simulink model "hybrid_pv_wind_feeder"  (R2024b)
settings: Solver=FixedStepDiscrete  StartTime=0.0  StopTime=1.0  FixedStep=P.Ts  RelTol=1e-3
model workspace (MAT data in the model file):
  P : object (value not decoded)
symbols that are objects in the model workspace (value not decoded): P
undefined symbols (not defined in the file): DiscIntNeverNeededParam
libraries: spsThreePhaseSeriesRLCBranchLib x28, spsSeriesRLCBranchLib x14, spsThreePhaseParallelRLCLoadLib x12, spsIGBTDiodeLib x8, slpidlib x7, spsThreePhaseBreakerLib x6, simulink x4, spsGroundLib x4, spsThreePhaseVIMeasurementLib x4, spsControlledCurrentSourceLib x3, spsDiodeLib x2, spsAlphaBetaZerotodq0Lib x2
(part 1 of 2)
Description:
  | Hybrid PV-wind unit on the Pidari 400 V feeder (NEA, Janakpur DC).
  | Built by scripts/build_feeder_model.m from hybrid_pv_wind_islanding.slx and Real_model/nea_lv_feeder_data.m.
settings Model: LastModifiedBy=subas
settings SolverCC: AlgebraicLoopSolver=LineSearch
settings DataIOCC: ReturnWorkspaceOutputs=off
settings DebuggingCC: AlgebraicLoopMsg=none  ArithmeticOperatorsInVariantConditions=warning
settings ModelReferenceCC: EnableRefExpFcnMdlSchedulingChecks=on
settings SFSimCC: SimUseLocalCustomCode=off  CustomCodeUndefinedFunction=UseInterfaceOnly
settings RTWCC: RTWUseLocalCustomCode=off  GPUComputeCapability=3.5

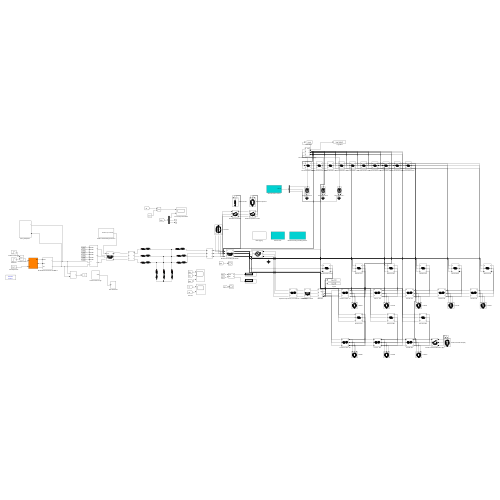
[thumbnail: Simulink's stored preview of the top-level diagram]
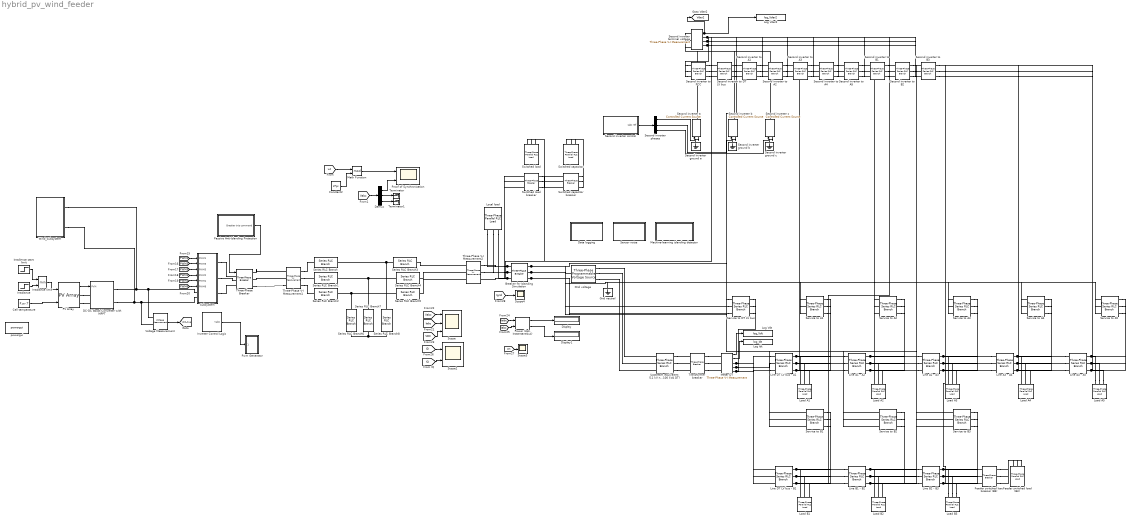
== system hybrid_pv_wind_feeder ==
  Breaker for Islanding Simulation : spsThreePhaseBreakerLib/Three-Phase Breaker  InitialState=closed  SwitchA=on  SwitchB=on  SwitchC=on  SwitchTimes=[P.tIsland]  External=off  BreakerResistance=0.01  SnubberResistance=1e6  SnubberCapacitance=inf  Measurements=None
  Cell temperature : Constant  Value=P.pv.T
  Constant2 : Constant  Value=2*pi
  DC-DC Boost Converter with MPPT : Subsystem
  Data logging : Subsystem
  Demux : Demux  Outputs=3
  Display : Display
  Display1 : Display
  Feeder switched load (B3) : spsThreePhaseParallelRLCLoadLib/Three-Phase Parallel RLC Load  LConnTagsString=A|B|C  Configuration=Y (grounded)  NominalVoltage=P.Vll  Vabc=[1e3 1e3 1e3]  Vabcp=[1e3 1e3 1e3]  NominalFrequency=P.fg  UnbalancedPower=off  ActivePower=P.feeder.swP  InductivePower=P.feeder.swQ  CapacitivePower=0  Pabc=[10e3 9e3 11e3]  QLabc=[100 90 110]  QCabc=[100 90 110]  Pabcp=[10e3 9e3 11e3]  QLabcp=[100 90 110]  QCabcp=[100 90 110]  Measurements=None  LoadType=constant Z
  Feeder switched load breaker (B3) : spsThreePhaseBreakerLib/Three-Phase Breaker  InitialState=open  SwitchA=on  SwitchB=on  SwitchC=on  SwitchTimes=[P.feeder.swT]  External=off  BreakerResistance=0.01  SnubberResistance=1e6  SnubberCapacitance=inf  Measurements=None
  Grid neutral : spsGroundLib/Ground  LConnTagsString=a
  Grid voltage : spsThreePhaseProgrammableVoltageSourceLib/Three-Phase Programmable Voltage Source  PositiveSequence=[P.feeder.Vsrc*P.Vll 0 P.fg]  VariationEntity=None  VariationType=Table of time-amplitude pairs  VariationTypeAlt=Step  VariationStep=P.event.step  VariationRate=P.event.rate  VariationMagnitude=0.3  VariationFrequency=2  VariationTiming=P.event.timing  VariationPhaseA=off  Amplitudes=P.event.amp  TimeValues=P.event.time  HarmonicGeneration=off  HarmonicA=P.grid.harmA  HarmonicB=P.grid.harmB  Timing=[0 1e6]  BusType=swing  Pref=0  Qref=0  Qmin=-inf  Qmax=inf
  Inverter Control Logic : Subsystem
  Irradiance : Step  Time=P.pv.tStep  Before=P.pv.G0  After=P.pv.G1  SampleTime=0
  Irradiance limit : MinMax  Inputs=2
  Irradiance start limit : Step  Time=P.pv.tStart  Before=P.pv.Gstart  After=1e4  SampleTime=0
  Line A1 - A2 : spsThreePhaseSeriesRLCBranchLib/Three-Phase Series RLC Branch  LConnTagsString=A|B|C  RConnTagsString=A|B|C  BranchType=RL  Resistance=P.feeder.lineR(2)  Inductance=P.feeder.lineL(2)  Capacitance=1e-6  Measurements=None
  Line A2 - A3 : spsThreePhaseSeriesRLCBranchLib/Three-Phase Series RLC Branch  LConnTagsString=A|B|C  RConnTagsString=A|B|C  BranchType=RL  Resistance=P.feeder.lineR(3)  Inductance=P.feeder.lineL(3)  Capacitance=1e-6  Measurements=None
  Line A3 - A4 : spsThreePhaseSeriesRLCBranchLib/Three-Phase Series RLC Branch  LConnTagsString=A|B|C  RConnTagsString=A|B|C  BranchType=RL  Resistance=P.feeder.lineR(4)  Inductance=P.feeder.lineL(4)  Capacitance=1e-6  Measurements=None
  Line A4 - A5 : spsThreePhaseSeriesRLCBranchLib/Three-Phase Series RLC Branch  LConnTagsString=A|B|C  RConnTagsString=A|B|C  BranchType=RL  Resistance=P.feeder.lineR(5)  Inductance=P.feeder.lineL(5)  Capacitance=1e-6  Measurements=None
  Line B1 - B2 : spsThreePhaseSeriesRLCBranchLib/Three-Phase Series RLC Branch  LConnTagsString=A|B|C  RConnTagsString=A|B|C  BranchType=RL  Resistance=P.feeder.lineR(7)  Inductance=P.feeder.lineL(7)  Capacitance=1e-6  Measurements=None
  Line B2 - B3 : spsThreePhaseSeriesRLCBranchLib/Three-Phase Series RLC Branch  LConnTagsString=A|B|C  RConnTagsString=A|B|C  BranchType=RL  Resistance=P.feeder.lineR(8)  Inductance=P.feeder.lineL(8)  Capacitance=1e-6  Measurements=None
  Line DT LV bus - A1 : spsThreePhaseSeriesRLCBranchLib/Three-Phase Series RLC Branch  LConnTagsString=A|B|C  RConnTagsString=A|B|C  BranchType=RL  Resistance=P.feeder.lineR(1)  Inductance=P.feeder.lineL(1)  Capacitance=1e-6  Measurements=None
  Line DT LV bus - B1 : spsThreePhaseSeriesRLCBranchLib/Three-Phase Series RLC Branch  LConnTagsString=A|B|C  RConnTagsString=A|B|C  BranchType=RL  Resistance=P.feeder.lineR(6)  Inductance=P.feeder.lineL(6)  Capacitance=1e-6  Measurements=None
  Load A1 : spsThreePhaseParallelRLCLoadLib/Three-Phase Parallel RLC Load  LConnTagsString=A|B|C  Configuration=Y (grounded)  NominalVoltage=P.Vll  Vabc=[1e3 1e3 1e3]  Vabcp=[1e3 1e3 1e3]  NominalFrequency=P.fg  UnbalancedPower=off  ActivePower=P.feeder.loadP(2)  InductivePower=P.feeder.loadQL(2)  CapacitivePower=0  Pabc=[10e3 9e3 11e3]  QLabc=[100 90 110]  QCabc=[100 90 110]  Pabcp=[10e3 9e3 11e3]  QLabcp=[100 90 110]  QCabcp=[100 90 110]  Measurements=None  LoadType=constant Z
  Load A2 : spsThreePhaseParallelRLCLoadLib/Three-Phase Parallel RLC Load  LConnTagsString=A|B|C  Configuration=Y (grounded)  NominalVoltage=P.Vll  Vabc=[1e3 1e3 1e3]  Vabcp=[1e3 1e3 1e3]  NominalFrequency=P.fg  UnbalancedPower=off  ActivePower=P.feeder.loadP(3)  InductivePower=P.feeder.loadQL(3)  CapacitivePower=0  Pabc=[10e3 9e3 11e3]  QLabc=[100 90 110]  QCabc=[100 90 110]  Pabcp=[10e3 9e3 11e3]  QLabcp=[100 90 110]  QCabcp=[100 90 110]  Measurements=None  LoadType=constant Z
  Load A3 : spsThreePhaseParallelRLCLoadLib/Three-Phase Parallel RLC Load  LConnTagsString=A|B|C  Configuration=Y (grounded)  NominalVoltage=P.Vll  Vabc=[1e3 1e3 1e3]  Vabcp=[1e3 1e3 1e3]  NominalFrequency=P.fg  UnbalancedPower=off  ActivePower=P.feeder.loadP(4)  InductivePower=P.feeder.loadQL(4)  CapacitivePower=0  Pabc=[10e3 9e3 11e3]  QLabc=[100 90 110]  QCabc=[100 90 110]  Pabcp=[10e3 9e3 11e3]  QLabcp=[100 90 110]  QCabcp=[100 90 110]  Measurements=None  LoadType=constant Z
  Load A4 : spsThreePhaseParallelRLCLoadLib/Three-Phase Parallel RLC Load  LConnTagsString=A|B|C  Configuration=Y (grounded)  NominalVoltage=P.Vll  Vabc=[1e3 1e3 1e3]  Vabcp=[1e3 1e3 1e3]  NominalFrequency=P.fg  UnbalancedPower=off  ActivePower=P.feeder.loadP(5)  InductivePower=P.feeder.loadQL(5)  CapacitivePower=0  Pabc=[10e3 9e3 11e3]  QLabc=[100 90 110]  QCabc=[100 90 110]  Pabcp=[10e3 9e3 11e3]  QLabcp=[100 90 110]  QCabcp=[100 90 110]  Measurements=None  LoadType=constant Z
  Load A5 : spsThreePhaseParallelRLCLoadLib/Three-Phase Parallel RLC Load  LConnTagsString=A|B|C  Configuration=Y (grounded)  NominalVoltage=P.Vll  Vabc=[1e3 1e3 1e3]  Vabcp=[1e3 1e3 1e3]  NominalFrequency=P.fg  UnbalancedPower=off  ActivePower=P.feeder.loadP(6)  InductivePower=P.feeder.loadQL(6)  CapacitivePower=0  Pabc=[10e3 9e3 11e3]  QLabc=[100 90 110]  QCabc=[100 90 110]  Pabcp=[10e3 9e3 11e3]  QLabcp=[100 90 110]  QCabcp=[100 90 110]  Measurements=None  LoadType=constant Z
  Load B1 : spsThreePhaseParallelRLCLoadLib/Three-Phase Parallel RLC Load  LConnTagsString=A|B|C  Configuration=Y (grounded)  NominalVoltage=P.Vll  Vabc=[1e3 1e3 1e3]  Vabcp=[1e3 1e3 1e3]  NominalFrequency=P.fg  UnbalancedPower=off  ActivePower=P.feeder.loadP(7)  InductivePower=P.feeder.loadQL(7)  CapacitivePower=0  Pabc=[10e3 9e3 11e3]  QLabc=[100 90 110]  QCabc=[100 90 110]  Pabcp=[10e3 9e3 11e3]  QLabcp=[100 90 110]  QCabcp=[100 90 110]  Measurements=None  LoadType=constant Z
  Load B2 : spsThreePhaseParallelRLCLoadLib/Three-Phase Parallel RLC Load  LConnTagsString=A|B|C  Configuration=Y (grounded)  NominalVoltage=P.Vll  Vabc=[1e3 1e3 1e3]  Vabcp=[1e3 1e3 1e3]  NominalFrequency=P.fg  UnbalancedPower=off  ActivePower=P.feeder.loadP(8)  InductivePower=P.feeder.loadQL(8)  CapacitivePower=0  Pabc=[10e3 9e3 11e3]  QLabc=[100 90 110]  QCabc=[100 90 110]  Pabcp=[10e3 9e3 11e3]  QLabcp=[100 90 110]  QCabcp=[100 90 110]  Measurements=None  LoadType=constant Z
  Load B3 : spsThreePhaseParallelRLCLoadLib/Three-Phase Parallel RLC Load  LConnTagsString=A|B|C  Configuration=Y (grounded)  NominalVoltage=P.Vll  Vabc=[1e3 1e3 1e3]  Vabcp=[1e3 1e3 1e3]  NominalFrequency=P.fg  UnbalancedPower=off  ActivePower=P.feeder.loadP(9)  InductivePower=P.feeder.loadQL(9)  CapacitivePower=0  Pabc=[10e3 9e3 11e3]  QLabc=[100 90 110]  QCabc=[100 90 110]  Pabcp=[10e3 9e3 11e3]  QLabcp=[100 90 110]  QCabcp=[100 90 110]  Measurements=None  LoadType=constant Z
  Local load : spsThreePhaseParallelRLCLoadLib/Three-Phase Parallel RLC Load  LConnTagsString=A|B|C  Configuration=Y (grounded)  NominalVoltage=P.Vll  Vabc=[1e3 1e3 1e3]  Vabcp=[1e3 1e3 1e3]  NominalFrequency=P.fg  UnbalancedPower=off  ActivePower=P.load.P  InductivePower=P.load.QL  CapacitivePower=P.load.QC  Pabc=[10e3 9e3 11e3]  QLabc=[100 90 110]  QCabc=[100 90 110]  Pabcp=[10e3 9e3 11e3]  QLabcp=[100 90 110]  QCabcp=[100 90 110]  Measurements=None  LoadType=constant Z
  Log Idt : ToWorkspace  VariableName=log_Idt  SaveFormat=Timeseries  SampleTime=-1
      settings: Decimation=P.logDecim
  Log Vder2 : ToWorkspace  VariableName=log_Vder2  SaveFormat=Timeseries  SampleTime=-1
      settings: Decimation=P.logDecim
  Log Vdt : ToWorkspace  VariableName=log_Vdt  SaveFormat=Timeseries  SampleTime=-1
      settings: Decimation=P.logDecim
  Machine-learning islanding detector : Subsystem
  Math Function : Math  Operator=mod  SignedPower=on
  Meter DT : spsThreePhaseVIMeasurementLib/Three-Phase V-I Measurement  VoltageMeasurement=phase-to-ground  SetLabelV=off  LabelV=Vabc  Vpu=off  VpuLL=off  CurrentMeasurement=yes  SetLabelI=off  LabelI=Iabc  Ipu=off  Pbase=100e6  Vbase=500e3  OutputType=Complex  PhasorSimulation=off  PSBequivalent=0
  PV Array : spsPVArrayLib/PV Array  Npar=P.pv.Npar  Nser=P.pv.Nser  PlotType=array @ 1000 W/m2 & specified temperatures  S_vec="[ 1000  500  100 ]"  Temp_C_vec="[ 45 25  ]"  ModuleName=User-defined  PlotWhenSelected=off  Pm=213.15  Ncell=60  Voc=36.3  Isc=7.84  Vm=29  Im=7.35  beta_Voc_pc=-0.36099  alpha_Isc_pc=0.102  beta_Voc=-0.13104  alpha_Isc=0.0079968  IL=7.8654  I0=2.9273e-10  nI=0.98119  Rsh=313.0553  Rs=0.39381  RobustModel=off  RobustCellTemperature=313.3991  BAL=on  Tc=1e-6  Tfilter=5e-5
  Passive Anti-Islanding Protection : Subsystem
  "Power (3ph, Instantaneous)" : spsPower3phInstantaneousLib/Power (3ph, Instantaneous)
  Proof of Synchronization : Scope  NumInputPorts=2
  "Pwm Generator " : Subsystem
  Scope : Scope  NumInputPorts=3
  Scope2 : Scope  NumInputPorts=2
  Scope3 : Scope
  Scope4 : Scope
  Second inverter a : spsControlledCurrentSourceLib/Controlled Current Source  Initialize=off  Source_Type=AC  Amplitude=0  Phase=0  Frequency=0  Measurements=None
  Second inverter b : spsControlledCurrentSourceLib/Controlled Current Source  Initialize=off  Source_Type=AC  Amplitude=0  Phase=0  Frequency=0  Measurements=None
  Second inverter c : spsControlledCurrentSourceLib/Controlled Current Source  Initialize=off  Source_Type=AC  Amplitude=0  Phase=0  Frequency=0  Measurements=None
  Second inverter control : Subsystem
  Second inverter ground a : spsGroundLib/Ground  LConnTagsString=a
  Second inverter ground b : spsGroundLib/Ground  LConnTagsString=a
  Second inverter ground c : spsGroundLib/Ground  LConnTagsString=a
  Second inverter phases : Demux  Outputs=3
  Second inverter terminal voltage : spsThreePhaseVIMeasurementLib/Three-Phase V-I Measurement  VoltageMeasurement=phase-to-ground  SetLabelV=off  LabelV=Vabc  Vpu=off  VpuLL=off  CurrentMeasurement=no  SetLabelI=off  LabelI=Iabc  Ipu=off  Pbase=100e6  Vbase=500e3  OutputType=Complex  PhasorSimulation=off  PSBequivalent=0
  Second inverter to A1 : spsThreePhaseSeriesRLCBranchLib/Three-Phase Series RLC Branch  LConnTagsString=A|B|C  RConnTagsString=A|B|C  BranchType=R  Resistance=P.feeder.rDer2(3)  Inductance=1e-3  Capacitance=1e-6  Measurements=None
  Second inverter to A2 : spsThreePhaseSeriesRLCBranchLib/Three-Phase Series RLC Branch  LConnTagsString=A|B|C  RConnTagsString=A|B|C  BranchType=R  Resistance=P.feeder.rDer2(4)  Inductance=1e-3  Capacitance=1e-6  Measurements=None
  Second inverter to A3 : spsThreePhaseSeriesRLCBranchLib/Three-Phase Series RLC Branch  LConnTagsString=A|B|C  RConnTagsString=A|B|C  BranchType=R  Resistance=P.feeder.rDer2(5)  Inductance=1e-3  Capacitance=1e-6  Measurements=None
  Second inverter to A4 : spsThreePhaseSeriesRLCBranchLib/Three-Phase Series RLC Branch  LConnTagsString=A|B|C  RConnTagsString=A|B|C  BranchType=R  Resistance=P.feeder.rDer2(6)  Inductance=1e-3  Capacitance=1e-6  Measurements=None
  Second inverter to A5 : spsThreePhaseSeriesRLCBranchLib/Three-Phase Series RLC Branch  LConnTagsString=A|B|C  RConnTagsString=A|B|C  BranchType=R  Resistance=P.feeder.rDer2(7)  Inductance=1e-3  Capacitance=1e-6  Measurements=None
  Second inverter to B1 : spsThreePhaseSeriesRLCBranchLib/Three-Phase Series RLC Branch  LConnTagsString=A|B|C  RConnTagsString=A|B|C  BranchType=R  Resistance=P.feeder.rDer2(8)  Inductance=1e-3  Capacitance=1e-6  Measurements=None
  Second inverter to B2 : spsThreePhaseSeriesRLCBranchLib/Three-Phase Series RLC Branch  LConnTagsString=A|B|C  RConnTagsString=A|B|C  BranchType=R  Resistance=P.feeder.rDer2(9)  Inductance=1e-3  Capacitance=1e-6  Measurements=None
  Second inverter to B3 : spsThreePhaseSeriesRLCBranchLib/Three-Phase Series RLC Branch  LConnTagsString=A|B|C  RConnTagsString=A|B|C  BranchType=R  Resistance=P.feeder.rDer2(10)  Inductance=1e-3  Capacitance=1e-6  Measurements=None
  Second inverter to DT LV bus : spsThreePhaseSeriesRLCBranchLib/Three-Phase Series RLC Branch  LConnTagsString=A|B|C  RConnTagsString=A|B|C  BranchType=R  Resistance=P.feeder.rDer2(2)  Inductance=1e-3  Capacitance=1e-6  Measurements=None
  Second inverter to PCC : spsThreePhaseSeriesRLCBranchLib/Three-Phase Series RLC Branch  LConnTagsString=A|B|C  RConnTagsString=A|B|C  BranchType=R  Resistance=P.feeder.rDer2(1)  Inductance=1e-3  Capacitance=1e-6  Measurements=None
  Sensor noise : Subsystem
  Series RLC Branch : spsSeriesRLCBranchLib/Series RLC Branch  LConnTagsString=__new0  RConnTagsString=__new0  BranchType=RL  Resistance=P.lcl.R1  Inductance=P.lcl.L1  SetiL0=off  InitialCurrent=0  Capacitance=1e-6  Setx0=off  InitialVoltage=0  Measurements=None
  Series RLC Branch1 : spsSeriesRLCBranchLib/Series RLC Branch  LConnTagsString=__new0  RConnTagsString=__new0  BranchType=RL  Resistance=P.lcl.R1  Inductance=P.lcl.L1  SetiL0=off  InitialCurrent=0  Capacitance=1e-6  Setx0=off  InitialVoltage=0  Measurements=None
  Series RLC Branch2 : spsSeriesRLCBranchLib/Series RLC Branch  LConnTagsString=__new0  RConnTagsString=__new0  BranchType=RL  Resistance=P.lcl.R1  Inductance=P.lcl.L1  SetiL0=off  InitialCurrent=0  Capacitance=1e-6  Setx0=off  InitialVoltage=0  Measurements=None
  Series RLC Branch3 : spsSeriesRLCBranchLib/Series RLC Branch  LConnTagsString=__new0  RConnTagsString=__new0  BranchType=RL  Resistance=P.lcl.R2  Inductance=P.lcl.L2  SetiL0=off  InitialCurrent=10  Capacitance=1e-6  Setx0=off  InitialVoltage=0  Measurements=None
  Series RLC Branch4 : spsSeriesRLCBranchLib/Series RLC Branch  LConnTagsString=__new0  RConnTagsString=__new0  BranchType=RL  Resistance=P.lcl.R2  Inductance=P.lcl.L2  SetiL0=off  InitialCurrent=10  Capacitance=1e-6  Setx0=off  InitialVoltage=0  Measurements=None
  Series RLC Branch5 : spsSeriesRLCBranchLib/Series RLC Branch  LConnTagsString=__new0  RConnTagsString=__new0  BranchType=RL  Resistance=P.lcl.R2  Inductance=P.lcl.L2  SetiL0=off  InitialCurrent=10  Capacitance=1e-6  Setx0=off  InitialVoltage=0  Measurements=None
  Series RLC Branch6 : spsSeriesRLCBranchLib/Series RLC Branch  LConnTagsString=__new0  RConnTagsString=__new0  BranchType=RC  Resistance=P.lcl.Rd  Inductance=1000e-3  SetiL0=off  InitialCurrent=0  Capacitance=P.lcl.Cf  Setx0=off  InitialVoltage=0  Measurements=None
  Series RLC Branch7 : spsSeriesRLCBranchLib/Series RLC Branch  LConnTagsString=__new0  RConnTagsString=__new0  BranchType=RC  Resistance=P.lcl.Rd  Inductance=1000e-3  SetiL0=off  InitialCurrent=0  Capacitance=P.lcl.Cf  Setx0=off  InitialVoltage=0  Measurements=None
  Series RLC Branch8 : spsSeriesRLCBranchLib/Series RLC Branch  LConnTagsString=__new0  RConnTagsString=__new0  BranchType=RC  Resistance=P.lcl.Rd  Inductance=1000e-3  SetiL0=off  InitialCurrent=0  Capacitance=P.lcl.Cf  Setx0=off  InitialVoltage=0  Measurements=None
  Service to A1 : spsThreePhaseSeriesRLCBranchLib/Three-Phase Series RLC Branch  LConnTagsString=A|B|C  RConnTagsString=A|B|C  BranchType=R  Resistance=P.feeder.rConn(2)  Inductance=1e-3  Capacitance=1e-6  Measurements=None
  Service to A2 : spsThreePhaseSeriesRLCBranchLib/Three-Phase Series RLC Branch  LConnTagsString=A|B|C  RConnTagsString=A|B|C  BranchType=R  Resistance=P.feeder.rConn(3)  Inductance=1e-3  Capacitance=1e-6  Measurements=None
  Service to A3 : spsThreePhaseSeriesRLCBranchLib/Three-Phase Series RLC Branch  LConnTagsString=A|B|C  RConnTagsString=A|B|C  BranchType=R  Resistance=P.feeder.rConn(4)  Inductance=1e-3  Capacitance=1e-6  Measurements=None
  Service to A4 : spsThreePhaseSeriesRLCBranchLib/Three-Phase Series RLC Branch  LConnTagsString=A|B|C  RConnTagsString=A|B|C  BranchType=R  Resistance=P.feeder.rConn(5)  Inductance=1e-3  Capacitance=1e-6  Measurements=None
  Service to A5 : spsThreePhaseSeriesRLCBranchLib/Three-Phase Series RLC Branch  LConnTagsString=A|B|C  RConnTagsString=A|B|C  BranchType=R  Resistance=P.feeder.rConn(6)  Inductance=1e-3  Capacitance=1e-6  Measurements=None
  Service to B1 : spsThreePhaseSeriesRLCBranchLib/Three-Phase Series RLC Branch  LConnTagsString=A|B|C  RConnTagsString=A|B|C  BranchType=R  Resistance=P.feeder.rConn(7)  Inductance=1e-3  Capacitance=1e-6  Measurements=None
  Service to B2 : spsThreePhaseSeriesRLCBranchLib/Three-Phase Series RLC Branch  LConnTagsString=A|B|C  RConnTagsString=A|B|C  BranchType=R  Resistance=P.feeder.rConn(8)  Inductance=1e-3  Capacitance=1e-6  Measurements=None
  Service to B3 : spsThreePhaseSeriesRLCBranchLib/Three-Phase Series RLC Branch  LConnTagsString=A|B|C  RConnTagsString=A|B|C  BranchType=R  Resistance=P.feeder.rConn(9)  Inductance=1e-3  Capacitance=1e-6  Measurements=None
  Service to DT LV bus : spsThreePhaseSeriesRLCBranchLib/Three-Phase Series RLC Branch  LConnTagsString=A|B|C  RConnTagsString=A|B|C  BranchType=R  Resistance=P.feeder.rConn(1)  Inductance=1e-3  Capacitance=1e-6  Measurements=None
  Subsystem : Subsystem
  Switched capacitor : spsThreePhaseParallelRLCLoadLib/Three-Phase Parallel RLC Load  LConnTagsString=A|B|C  Configuration=Y (grounded)  NominalVoltage=P.Vll  Vabc=[1e3 1e3 1e3]  Vabcp=[1e3 1e3 1e3]  NominalFrequency=P.fg  UnbalancedPower=off  ActivePower=1  InductivePower=0  CapacitivePower=P.event.capQ  Pabc=[10e3 9e3 11e3]  QLabc=[100 90 110]  QCabc=[100 90 110]  Pabcp=[10e3 9e3 11e3]  QLabcp=[100 90 110]  QCabcp=[100 90 110]  Measurements=None  LoadType=constant Z
  Switched capacitor breaker : spsThreePhaseBreakerLib/Three-Phase Breaker  InitialState=open  SwitchA=on  SwitchB=on  SwitchC=on  SwitchTimes=[P.event.capT]  External=off  BreakerResistance=0.01  SnubberResistance=1e6  SnubberCapacitance=inf  Measurements=None
  Switched load : spsThreePhaseParallelRLCLoadLib/Three-Phase Parallel RLC Load  LConnTagsString=A|B|C  Configuration=Y (grounded)  NominalVoltage=P.Vll  Vabc=[1e3 1e3 1e3]  Vabcp=[1e3 1e3 1e3]  NominalFrequency=P.fg  UnbalancedPower=off  ActivePower=P.event.loadP  InductivePower=0  CapacitivePower=0  Pabc=[10e3 9e3 11e3]  QLabc=[100 90 110]  QCabc=[100 90 110]  Pabcp=[10e3 9e3 11e3]  QLabcp=[100 90 110]  QCabcp=[100 90 110]  Measurements=None  LoadType=constant Z
  Switched load breaker : spsThreePhaseBreakerLib/Three-Phase Breaker  InitialState=open  SwitchA=on  SwitchB=on  SwitchC=on  SwitchTimes=[P.event.loadT]  External=off  BreakerResistance=0.01  SnubberResistance=1e6  SnubberCapacitance=inf  Measurements=None
  Terminator : Terminator
  Terminator1 : Terminator
  Three-Phase V-I Measurement1 : spsThreePhaseVIMeasurementLib/Three-Phase V-I Measurement  VoltageMeasurement=no  SetLabelV=off  LabelV=Vabc  Vpu=off  VpuLL=off  CurrentMeasurement=yes  SetLabelI=on  LabelI=Iabc_true  Ipu=off  Pbase=100e6  Vbase=500e3  OutputType=Complex  PhasorSimulation=off  PSBequivalent=0
  Three-Phase V-I Measurement2 : spsThreePhaseVIMeasurementLib/Three-Phase V-I Measurement  VoltageMeasurement=phase-to-ground  SetLabelV=on  LabelV=Vabc_true  Vpu=off  VpuLL=off  CurrentMeasurement=yes  SetLabelI=on  LabelI=Igrid_true  Ipu=off  Pbase=100e6  Vbase=500e3  OutputType=Complex  PhasorSimulation=off  PSBequivalent=0
  Three-Phase Breaker : spsThreePhaseBreakerLib/Three-Phase Breaker  InitialState=closed  SwitchA=on  SwitchB=on  SwitchC=on  SwitchTimes=[9999]  External=on  BreakerResistance=0.01  SnubberResistance=1e6  SnubberCapacitance=inf  Measurements=None
  Transformer breaker : spsThreePhaseBreakerLib/Three-Phase Breaker  InitialState=closed  SwitchA=on  SwitchB=on  SwitchC=on  SwitchTimes=[P.feeder.tIsland]  External=off  BreakerResistance=0.01  SnubberResistance=1e6  SnubberCapacitance=inf  Measurements=None
  Upstream equivalent (11 kV network + 100 kVA DT) : spsThreePhaseSeriesRLCBranchLib/Three-Phase Series RLC Branch  LConnTagsString=A|B|C  RConnTagsString=A|B|C  BranchType=RL  Resistance=P.feeder.Rsrc  Inductance=P.feeder.Lsrc  Capacitance=1e-6  Measurements=None
  Voltage Measurement : spsVoltageMeasurementLib/Voltage Measurement  PhasorSimulation=off  OutputType=Complex  PSBequivalent=0
  Wind_Subsystem : Subsystem
  powergui : spspowerguiLib/powergui  Priority=1  SimulationMode=Discrete  SampleTime=P.Ts  frequency=60  Iterations=50  frequencyindice=0  Pbase=100e6  ErrMax=1e-4  UnitsV=kV  UnitsW=MW  buscounter=0  FunctionMessages=off  echomessages=off  EnableUseOfTLC=off  CurrentSourceSwitches=off  DisableSnubberDevices=off  DisableRonSwitches=off  DisableVfSwitches=off  DisplayEquations=off  AutomaticDiscreteSolvers=off  SolverType=Tustin/Backward Euler (TBE)  Interpol=off  ExternalGateDelay=off  methode=off  Ts=100  x0status=blocks  SPID=off  SwTol=0  HookPort=off  NonlinearTolerance=1e-4  nMaxIteration=100  ContinueOnMaxIteration=off  RestoreLinks=warning  ResistiveCurrentMeasurement=off  Frange=[0:2:500]  Ylog=off  Xlog=on  ShowGrid=off  save=off  variable=ZData  structure=Grid_current  ZoomFFT=off  StartTime=0.4  cycles=5  DisplayStyle=1  fundamental=50  FreqAxis=off  MaxFrequency=1000  frequencyindicesteady=1  RmsSteady=1  display=off
  tag scope: VDC_true=global, Vder2=global
  wires:
  Voltage Measurement/1 -> [VDC_true]
  [PWM6] -> Subsystem/6(PWM6)
  [PWM1] -> Subsystem/1(PWM1)
  "Power (3ph, Instantaneous)"/1 -> Display/1
  PV Array/1 -> DC-DC Boost Converter with MPPT/1("PVM ")
  [Iabc] -> "Power (3ph, Instantaneous)"/2
  [PWM3] -> Subsystem/2(PWM3)
  [Igrid] -> Scope4/1
  Inverter Control Logic/1(Vabc) -> "Pwm Generator "/1(1)
  [PWM4] -> Subsystem/5(PWM4)
  [Vabc] -> Scope/1
  [Vabc] -> "Power (3ph, Instantaneous)"/1
  [ID] -> Scope2/1
  "Power (3ph, Instantaneous)"/2 -> Display1/1
  [wt] -> Scope3/1
  [PWM2] -> Subsystem/4(PWM2)
  [VDC] -> Scope/3
  [PWM5] -> Subsystem/3(PWM5)
  [Iabc] -> Scope/2
  Passive Anti-Islanding Protection/1("Breaker trip command ") -> Three-Phase Breaker/1
  Demux/1 -> Proof of Synchronization/2
  Demux/2 -> Terminator/1
  Constant2/1 -> Math Function/2
  [wt] -> Math Function/1
  Math Function/1 -> Proof of Synchronization/1
  [Vabc] -> Demux/1
  Demux/3 -> Terminator1/1
  Irradiance/1 -> Irradiance limit/2
  Irradiance start limit/1 -> Irradiance limit/1
  Irradiance limit/1 -> PV Array/1
  Cell temperature/1 -> PV Array/2
  Second inverter control/1(Iabc ref) -> Second inverter phases/1
  Second inverter phases/1 -> Second inverter a/1
  Second inverter phases/2 -> Second inverter b/1
  Second inverter phases/3 -> Second inverter c/1
  [IQ] -> Scope2/2
  Meter DT/1 -> Log Vdt/1
  Meter DT/2 -> Log Idt/1
  Second inverter terminal voltage/1 -> [Vder2], Log Vder2/1
  connections:
  Series RLC Branch7/RConn1 -- Series RLC Branch8/RConn1 -- Series RLC Branch6/RConn1
  Series RLC Branch8/LConn1 -- Series RLC Branch/RConn1 -- Series RLC Branch3/LConn1
  Series RLC Branch7/LConn1 -- Series RLC Branch1/RConn1 -- Series RLC Branch4/LConn1
  Series RLC Branch6/LConn1 -- Series RLC Branch2/RConn1 -- Series RLC Branch5/LConn1
  PV Array/RConn1 -- DC-DC Boost Converter with MPPT/LConn1
  Three-Phase V-I Measurement1/RConn3 -- Series RLC Branch2/LConn1
  Three-Phase V-I Measurement1/RConn1 -- Series RLC Branch/LConn1
  PV Array/RConn2 -- DC-DC Boost Converter with MPPT/LConn2
  Three-Phase V-I Measurement1/RConn2 -- Series RLC Branch1/LConn1
  DC-DC Boost Converter with MPPT/RConn1 -- Wind_Subsystem/RConn1 -- Subsystem/LConn1 -- Voltage Measurement/LConn1
  DC-DC Boost Converter with MPPT/RConn2 -- Wind_Subsystem/RConn2 -- Subsystem/LConn2 -- Voltage Measurement/LConn2
  Subsystem/RConn1 -- Three-Phase Breaker/LConn1
  Subsystem/RConn2 -- Three-Phase Breaker/LConn2
  Subsystem/RConn3 -- Three-Phase Breaker/LConn3
  Three-Phase Breaker/RConn1 -- Three-Phase V-I Measurement1/LConn1
  Three-Phase V-I Measurement1/LConn2 -- Three-Phase Breaker/RConn2
  Three-Phase Breaker/RConn3 -- Three-Phase V-I Measurement1/LConn3
  Three-Phase V-I Measurement2/LConn1 -- Local load/LConn1 -- Switched load breaker/LConn1 -- Switched capacitor breaker/LConn1 -- Breaker for Islanding Simulation/LConn1 -- Second inverter to PCC/RConn1
  Three-Phase V-I Measurement2/LConn2 -- Local load/LConn2 -- Switched load breaker/LConn2 -- Switched capacitor breaker/LConn2 -- Breaker for Islanding Simulation/LConn2 -- Second inverter to PCC/RConn2
  Three-Phase V-I Measurement2/LConn3 -- Breaker for Islanding Simulation/LConn3 -- Local load/LConn3 -- Switched load breaker/LConn3 -- Switched capacitor breaker/LConn3 -- Second inverter to PCC/RConn3
  Series RLC Branch3/RConn1 -- Three-Phase V-I Measurement2/RConn1
  Series RLC Branch4/RConn1 -- Three-Phase V-I Measurement2/RConn2
  Series RLC Branch5/RConn1 -- Three-Phase V-I Measurement2/RConn3
  Grid voltage/LConn1 -- Grid neutral/LConn1
  Switched load breaker/RConn1 -- Switched load/LConn1
  Switched load breaker/RConn2 -- Switched load/LConn2
  Switched load breaker/RConn3 -- Switched load/LConn3
  Switched capacitor breaker/RConn1 -- Switched capacitor/LConn1
  Switched capacitor breaker/RConn2 -- Switched capacitor/LConn2
  Switched capacitor breaker/RConn3 -- Switched capacitor/LConn3
  Second inverter a/LConn1 -- Second inverter ground a/LConn1
  Second inverter b/LConn1 -- Second inverter ground b/LConn1
  Second inverter c/LConn1 -- Second inverter ground c/LConn1
  Grid voltage/RConn1 -- Upstream equivalent (11 kV network + 100 kVA DT)/LConn1
  Grid voltage/RConn2 -- Upstream equivalent (11 kV network + 100 kVA DT)/LConn2
  Grid voltage/RConn3 -- Upstream equivalent (11 kV network + 100 kVA DT)/LConn3
  Upstream equivalent (11 kV network + 100 kVA DT)/RConn1 -- Transformer breaker/LConn1
  Upstream equivalent (11 kV network + 100 kVA DT)/RConn2 -- Transformer breaker/LConn2
  Upstream equivalent (11 kV network + 100 kVA DT)/RConn3 -- Transformer breaker/LConn3
  Transformer breaker/RConn1 -- Meter DT/LConn1
  Transformer breaker/RConn2 -- Meter DT/LConn2
  Transformer breaker/RConn3 -- Meter DT/LConn3
  Line DT LV bus - A1/LConn1 -- Meter DT/RConn1 -- Line DT LV bus - B1/LConn1 -- Service to DT LV bus/RConn1 -- Second inverter to DT LV bus/RConn1
  Line DT LV bus - A1/LConn2 -- Meter DT/RConn2 -- Line DT LV bus - B1/LConn2 -- Service to DT LV bus/RConn2 -- Second inverter to DT LV bus/RConn2
  Line DT LV bus - A1/LConn3 -- Meter DT/RConn3 -- Line DT LV bus - B1/LConn3 -- Service to DT LV bus/RConn3 -- Second inverter to DT LV bus/RConn3
  Line A1 - A2/LConn1 -- Line DT LV bus - A1/RConn1 -- Load A1/LConn1 -- Service to A1/RConn1 -- Second inverter to A1/RConn1
  Line A1 - A2/LConn2 -- Line DT LV bus - A1/RConn2 -- Load A1/LConn2 -- Service to A1/RConn2 -- Second inverter to A1/RConn2
  Line A1 - A2/LConn3 -- Line DT LV bus - A1/RConn3 -- Load A1/LConn3 -- Service to A1/RConn3 -- Second inverter to A1/RConn3
  Line A2 - A3/LConn1 -- Line A1 - A2/RConn1 -- Load A2/LConn1 -- Service to A2/RConn1 -- Second inverter to A2/RConn1
  Line A2 - A3/LConn2 -- Line A1 - A2/RConn2 -- Load A2/LConn2 -- Service to A2/RConn2 -- Second inverter to A2/RConn2
  Line A2 - A3/LConn3 -- Line A1 - A2/RConn3 -- Load A2/LConn3 -- Service to A2/RConn3 -- Second inverter to A2/RConn3
  Line A3 - A4/LConn1 -- Line A2 - A3/RConn1 -- Load A3/LConn1 -- Service to A3/RConn1 -- Second inverter to A3/RConn1
  Line A3 - A4/LConn2 -- Line A2 - A3/RConn2 -- Load A3/LConn2 -- Service to A3/RConn2 -- Second inverter to A3/RConn2
  Line A3 - A4/LConn3 -- Line A2 - A3/RConn3 -- Load A3/LConn3 -- Service to A3/RConn3 -- Second inverter to A3/RConn3
  Line A4 - A5/LConn1 -- Line A3 - A4/RConn1 -- Load A4/LConn1 -- Service to A4/RConn1 -- Second inverter to A4/RConn1
  Line A4 - A5/LConn2 -- Line A3 - A4/RConn2 -- Load A4/LConn2 -- Service to A4/RConn2 -- Second inverter to A4/RConn2
  Line A4 - A5/LConn3 -- Line A3 - A4/RConn3 -- Load A4/LConn3 -- Service to A4/RConn3 -- Second inverter to A4/RConn3
  Line B1 - B2/LConn1 -- Line DT LV bus - B1/RConn1 -- Load B1/LConn1 -- Service to B1/RConn1 -- Second inverter to B1/RConn1
  Line B1 - B2/LConn2 -- Line DT LV bus - B1/RConn2 -- Load B1/LConn2 -- Service to B1/RConn2 -- Second inverter to B1/RConn2
  Line B1 - B2/LConn3 -- Line DT LV bus - B1/RConn3 -- Load B1/LConn3 -- Service to B1/RConn3 -- Second inverter to B1/RConn3
  Line B2 - B3/LConn1 -- Line B1 - B2/RConn1 -- Load B2/LConn1 -- Service to B2/RConn1 -- Second inverter to B2/RConn1
  Line B2 - B3/LConn2 -- Line B1 - B2/RConn2 -- Load B2/LConn2 -- Service to B2/RConn2 -- Second inverter to B2/RConn2
  Line B2 - B3/LConn3 -- Line B1 - B2/RConn3 -- Load B2/LConn3 -- Service to B2/RConn3 -- Second inverter to B2/RConn3
  Load A5/LConn1 -- Line A4 - A5/RConn1 -- Service to A5/RConn1 -- Second inverter to A5/RConn1
  Load A5/LConn2 -- Line A4 - A5/RConn2 -- Service to A5/RConn2 -- Second inverter to A5/RConn2
  Load A5/LConn3 -- Line A4 - A5/RConn3 -- Service to A5/RConn3 -- Second inverter to A5/RConn3
  Load B3/LConn1 -- Line B2 - B3/RConn1 -- Feeder switched load breaker (B3)/LConn1 -- Service to B3/RConn1 -- Second inverter to B3/RConn1
  Load B3/LConn2 -- Line B2 - B3/RConn2 -- Feeder switched load breaker (B3)/LConn2 -- Service to B3/RConn2 -- Second inverter to B3/RConn2
  Load B3/LConn3 -- Line B2 - B3/RConn3 -- Feeder switched load breaker (B3)/LConn3 -- Service to B3/RConn3 -- Second inverter to B3/RConn3
  Feeder switched load breaker (B3)/RConn1 -- Feeder switched load (B3)/LConn1
  Feeder switched load breaker (B3)/RConn2 -- Feeder switched load (B3)/LConn2
  Feeder switched load breaker (B3)/RConn3 -- Feeder switched load (B3)/LConn3
  Service to DT LV bus/LConn1 -- Breaker for Islanding Simulation/RConn1 -- Service to A1/LConn1 -- Service to A2/LConn1 -- Service to A3/LConn1 -- Service to A4/LConn1 -- Service to A5/LConn1 -- Service to B1/LConn1 -- Service to B2/LConn1 -- Service to B3/LConn1
  Service to DT LV bus/LConn2 -- Breaker for Islanding Simulation/RConn2 -- Service to A1/LConn2 -- Service to A2/LConn2 -- Service to A3/LConn2 -- Service to A4/LConn2 -- Service to A5/LConn2 -- Service to B1/LConn2 -- Service to B2/LConn2 -- Service to B3/LConn2
  Service to DT LV bus/LConn3 -- Breaker for Islanding Simulation/RConn3 -- Service to A1/LConn3 -- Service to A2/LConn3 -- Service to A3/LConn3 -- Service to A4/LConn3 -- Service to A5/LConn3 -- Service to B1/LConn3 -- Service to B2/LConn3 -- Service to B3/LConn3
  Second inverter a/RConn1 -- Second inverter terminal voltage/LConn1
  Second inverter b/RConn1 -- Second inverter terminal voltage/LConn2
  Second inverter c/RConn1 -- Second inverter terminal voltage/LConn3
  Second inverter to PCC/LConn1 -- Second inverter terminal voltage/RConn1 -- Second inverter to DT LV bus/LConn1 -- Second inverter to A1/LConn1 -- Second inverter to A2/LConn1 -- Second inverter to A3/LConn1 -- Second inverter to A4/LConn1 -- Second inverter to A5/LConn1 -- Second inverter to B1/LConn1 -- Second inverter to B2/LConn1 -- Second inverter to B3/LConn1
  Second inverter to PCC/LConn2 -- Second inverter terminal voltage/RConn2 -- Second inverter to DT LV bus/LConn2 -- Second inverter to A1/LConn2 -- Second inverter to A2/LConn2 -- Second inverter to A3/LConn2 -- Second inverter to A4/LConn2 -- Second inverter to A5/LConn2 -- Second inverter to B1/LConn2 -- Second inverter to B2/LConn2 -- Second inverter to B3/LConn2
  Second inverter to PCC/LConn3 -- Second inverter terminal voltage/RConn3 -- Second inverter to DT LV bus/LConn3 -- Second inverter to A1/LConn3 -- Second inverter to A2/LConn3 -- Second inverter to A3/LConn3 -- Second inverter to A4/LConn3 -- Second inverter to A5/LConn3 -- Second inverter to B1/LConn3 -- Second inverter to B2/LConn3 -- Second inverter to B3/LConn3

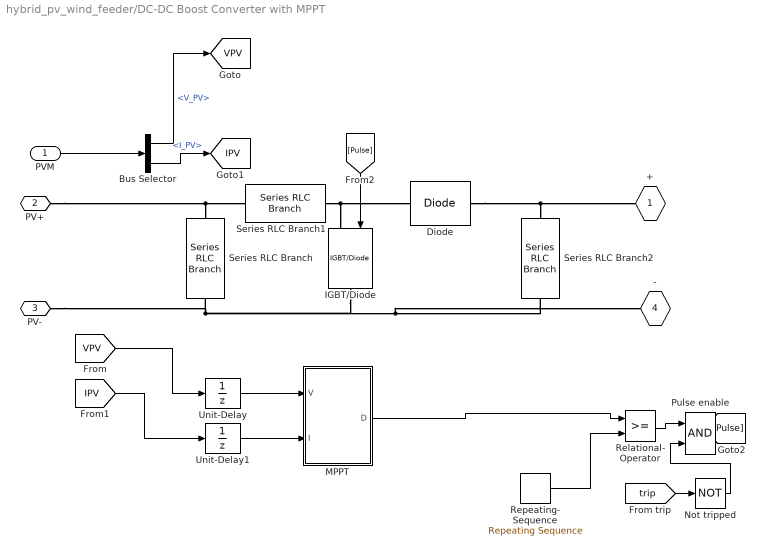
== system hybrid_pv_wind_feeder/DC-DC Boost Converter with MPPT ==
  "PVM " : Inport
  Bus Selector : BusSelector  OutputSignals=V_PV,I_PV
  Diode : spsDiodeLib/Diode  Ron=0.001  Lon=0  Vf=0.8  IC=0  UseSnubber=0  Rs=500  Cs=250e-9  Measurements=off
  IGBT/Diode : spsIGBTDiodeLib/IGBT//Diode  Ron=1e-3  Rs=1e5  Cs=inf  Measurements=off
  MPPT : MATLAB Function  TreatAsAtomicUnit=on
  Not tripped : Logic  Operator=NOT  AllPortsSameDT=off  OutDataTypeStr=boolean
  Pulse enable : Logic  AllPortsSameDT=off  OutDataTypeStr=boolean
  Relational- Operator : RelationalOperator  OutDataTypeStr=boolean  RndMeth=Simplest  InputSameDT=off
  Repeating- Sequence : simulink/Sources/Repeating Sequence  rep_seq_t=[0 0.0002]  rep_seq_y=[0 1]
  Series RLC Branch : spsSeriesRLCBranchLib/Series RLC Branch  LConnTagsString=__new0  RConnTagsString=__new0  BranchType=RC  Resistance=1e-3  Inductance=1e-3  SetiL0=off  InitialCurrent=0  Capacitance=1000e-6  Setx0=off  InitialVoltage=0  Measurements=None
  Series RLC Branch1 : spsSeriesRLCBranchLib/Series RLC Branch  LConnTagsString=__new0  RConnTagsString=__new0  BranchType=L  Resistance=1e-3  Inductance=1.5e-3  SetiL0=off  InitialCurrent=0  Capacitance=1000e-6  Setx0=off  InitialVoltage=0  Measurements=None
  Series RLC Branch2 : spsSeriesRLCBranchLib/Series RLC Branch  LConnTagsString=__new0  RConnTagsString=__new0  BranchType=C  Resistance=1e-3  Inductance=1e-3  SetiL0=off  InitialCurrent=0  Capacitance=3227e-6  Setx0=on  InitialVoltage=P.Vdc  Measurements=None
  Unit-Delay : UnitDelay  SampleTime=P.pv.Tmppt  HasFrameUpgradeWarning=on
  Unit-Delay1 : UnitDelay  SampleTime=P.pv.Tmppt  HasFrameUpgradeWarning=on
  + : PMIOPort  Side=Right
  PV+ : PMIOPort  Port=2  Side=Left
  PV- : PMIOPort  Port=3  Side=Left
  - : PMIOPort  Port=4  Side=Right
  tag scope: IPV=global, VPV=global
  wires:
  [Pulse] -> IGBT/Diode/1
  Bus Selector/1 -> [VPV]  "<V_PV>"
  Bus Selector/2 -> [IPV]  "<I_PV>"
  "PVM "/1 -> Bus Selector/1
  [VPV] -> Unit-Delay/1
  Unit-Delay/1 -> MPPT/1(V)
  Repeating- Sequence/1 -> Relational- Operator/2
  Unit-Delay1/1 -> MPPT/2(I)
  [IPV] -> Unit-Delay1/1
  MPPT/1(D) -> Relational- Operator/1
  [trip] -> Not tripped/1
  Relational- Operator/1 -> Pulse enable/1
  Not tripped/1 -> Pulse enable/2
  Pulse enable/1 -> [Pulse]
  connections:
  Diode/RConn1 -- +/RConn1 -- Series RLC Branch2/LConn1
  Series RLC Branch/RConn1 -- PV-/RConn1 -- -/RConn1 -- Series RLC Branch2/RConn1 -- IGBT/Diode/RConn1
  Series RLC Branch1/LConn1 -- Diode/LConn1 -- IGBT/Diode/LConn1
  Series RLC Branch/LConn1 -- PV+/RConn1 -- Series RLC Branch1/RConn1

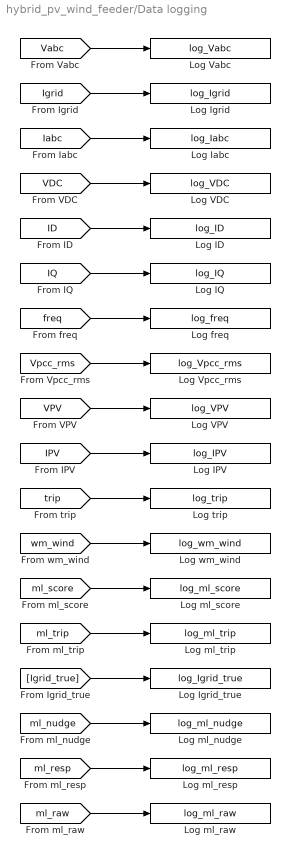
== system hybrid_pv_wind_feeder/Data logging ==
  Log ID : ToWorkspace  VariableName=log_ID  SaveFormat=Timeseries  SampleTime=-1
      settings: Decimation=P.logDecim
  Log IPV : ToWorkspace  VariableName=log_IPV  SaveFormat=Timeseries  SampleTime=-1
      settings: Decimation=P.logDecim
  Log IQ : ToWorkspace  VariableName=log_IQ  SaveFormat=Timeseries  SampleTime=-1
      settings: Decimation=P.logDecim
  Log Iabc : ToWorkspace  VariableName=log_Iabc  SaveFormat=Timeseries  SampleTime=-1
      settings: Decimation=P.logDecim
  Log Igrid : ToWorkspace  VariableName=log_Igrid  SaveFormat=Timeseries  SampleTime=-1
      settings: Decimation=P.logDecim
  Log Igrid_true : ToWorkspace  VariableName=log_Igrid_true  SaveFormat=Timeseries  SampleTime=-1
      settings: Decimation=P.logDecim
  Log VDC : ToWorkspace  VariableName=log_VDC  SaveFormat=Timeseries  SampleTime=-1
      settings: Decimation=P.logDecim
  Log VPV : ToWorkspace  VariableName=log_VPV  SaveFormat=Timeseries  SampleTime=-1
      settings: Decimation=P.logDecim
  Log Vabc : ToWorkspace  VariableName=log_Vabc  SaveFormat=Timeseries  SampleTime=-1
      settings: Decimation=P.logDecim
  Log Vpcc_rms : ToWorkspace  VariableName=log_Vpcc_rms  SaveFormat=Timeseries  SampleTime=-1
      settings: Decimation=P.logDecim
  Log freq : ToWorkspace  VariableName=log_freq  SaveFormat=Timeseries  SampleTime=-1
      settings: Decimation=P.logDecim
  Log ml_nudge : ToWorkspace  VariableName=log_ml_nudge  SaveFormat=Timeseries  SampleTime=-1
      settings: Decimation=P.logDecim
  Log ml_raw : ToWorkspace  VariableName=log_ml_raw  SaveFormat=Timeseries  SampleTime=-1
      settings: Decimation=P.logDecim
  Log ml_resp : ToWorkspace  VariableName=log_ml_resp  SaveFormat=Timeseries  SampleTime=-1
      settings: Decimation=P.logDecim
  Log ml_score : ToWorkspace  VariableName=log_ml_score  SaveFormat=Timeseries  SampleTime=-1
      settings: Decimation=P.logDecim
  Log ml_trip : ToWorkspace  VariableName=log_ml_trip  SaveFormat=Timeseries  SampleTime=-1
      settings: Decimation=P.logDecim
  Log trip : ToWorkspace  VariableName=log_trip  SaveFormat=Timeseries  SampleTime=-1
      settings: Decimation=P.logDecim
  Log wm_wind : ToWorkspace  VariableName=log_wm_wind  SaveFormat=Timeseries  SampleTime=-1
      settings: Decimation=P.logDecim
  wires:
  [Vabc] -> Log Vabc/1
  [Igrid] -> Log Igrid/1
  [Iabc] -> Log Iabc/1
  [VDC] -> Log VDC/1
  [ID] -> Log ID/1
  [IQ] -> Log IQ/1
  [freq] -> Log freq/1
  [Vpcc_rms] -> Log Vpcc_rms/1
  [VPV] -> Log VPV/1
  [IPV] -> Log IPV/1
  [trip] -> Log trip/1
  [wm_wind] -> Log wm_wind/1
  [ml_score] -> Log ml_score/1
  [ml_trip] -> Log ml_trip/1
  [Igrid_true] -> Log Igrid_true/1
  [ml_nudge] -> Log ml_nudge/1
  [ml_resp] -> Log ml_resp/1
  [ml_raw] -> Log ml_raw/1

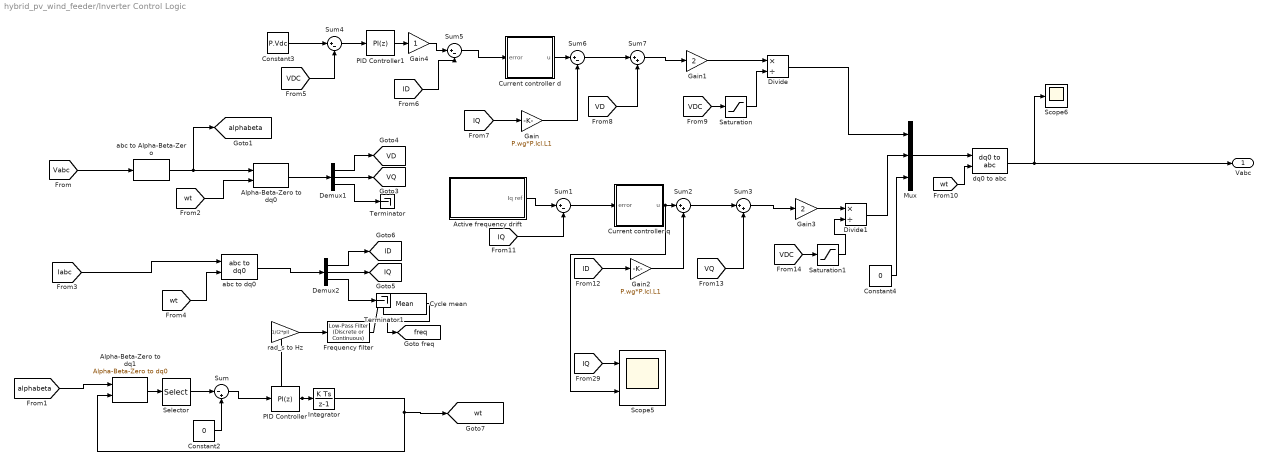
== system hybrid_pv_wind_feeder/Inverter Control Logic ==
  Active frequency drift : Subsystem
  Alpha-Beta-Zero to dq0 : spsAlphaBetaZerotodq0Lib/Alpha-Beta-Zero to dq0  Alignment=90 degrees behind phase A axis
  Alpha-Beta-Zero to dq1 : spsAlphaBetaZerotodq0Lib/Alpha-Beta-Zero to dq0  Alignment=90 degrees behind phase A axis
  Constant2 : Constant  Value=0
  Constant3 : Constant  Value=P.Vdc
  Constant4 : Constant  Value=0
  Current controller d : Subsystem
  Current controller q : Subsystem
  Cycle mean : spsMeanLib/Mean  Freq=P.fg  Vinit=P.fg  Ts=P.Ts
  Demux1 : Demux  Outputs=3
  Demux2 : Demux  Outputs=3
  Divide : Product  Inputs=*/
  Divide1 : Product  Inputs=*/
  Frequency filter : eeGeneralControl/Low-Pass Filter (Discrete or Continuous)  K=1  T=P.pll.Tf  B=inf  A=-inf  init_option=Inherited from block input  x0=0  Ts=-1
  Gain : Gain  Gain=P.wg*P.lcl.L1
  Gain1 : Gain  Gain=2
  Gain2 : Gain  Gain=P.wg*P.lcl.L1
  Gain3 : Gain  Gain=2
  Gain4 : Gain
  Integrator : DiscreteIntegrator  SampleTime=-1  ICPrevOutput=DiscIntNeverNeededParam  ICPrevScaledInput=DiscIntNeverNeededParam
  Mux : Mux  Inputs=3
  PID Controller : slpidlib/PID Controller  Controller=PI  Form=Parallel  TimeDomain=Discrete-time  UseExternalTs=off  SampleTime=-1  IntegratorMethod=Forward Euler  FilterMethod=Forward Euler  ControllerParametersSource=internal  P=P.pll.Kp  I=P.pll.Ki  UseKiTs=off  D=0  UseExternalDerivativeSource=off  N=100  UseFilter=on  TunerSelectOption=Transfer Function Based (PID Tuner App)  InitialConditionSource=internal  InitialConditionForIntegrator=P.wg  InitialConditionForFilter=0  DifferentiatorICPrevScaledInput=0  ExternalReset=none  TrackingMode=off  Kt=1  LimitOutput=off  SatLimitsSource=internal  UpperSaturationLimit=inf  LowerSaturationLimit=-inf  LinearizeAsGain=on  AntiWindupMode=none  Kb=1  LimitIntegrator=off  UpperIntegratorSaturationLimit=inf  LowerIntegratorSaturationLimit=-inf  POutMin=[]  POutMax=[]  IOutMin=[]  IOutMax=[]  DOutMin=[]  DOutMax=[]  NOutMin=[]  NOutMax=[]  SumOutMin=[]  SumOutMax=[]  SaturationOutMin=[]  SaturationOutMax=[]  PParamMin=[]  PParamMax=[]  IParamMin=[]  IParamMax=[]  DParamMin=[]  DParamMax=[]  NParamMin=[]  NParamMax=[]  KbParamMin=[]  KbParamMax=[]  KtParamMin=[]  KtParamMax=[]  KbOutMin=[]  KbOutMax=[]  KtOutMin=[]  KtOutMax=[]  IntegratorOutMin=[]  IntegratorOutMax=[]  FilterOutMin=[]  FilterOutMax=[]  SumI1OutMin=[]  SumI1OutMax=[]  SumI2OutMin=[]  SumI2OutMax=[]  SumI3OutMin=[]  SumI3OutMax=[]  SumI4OutMin=[]  SumI4OutMax=[]  SumDOutMin=[]  SumDOutMax=[]  DifferentiatorOutMin=[]  DifferentiatorOutMax=[]  FilterDiffOutCoefMin=[]  FilterDiffOutCoefMax=[]  ReciprocalOutMin=[]  ReciprocalOutMax=[]  SumDenOutMin=[]  SumDenOutMax=[]  SumNumOutMin=[]  SumNumOutMax=[]  DivideOutMin=[]  DivideOutMax=[]  UdiffTsProdOutMin=[]  UdiffTsProdOutMax=[]  NTsProdOutMin=[]  NTsProdOutMax=[]  UintegralTsProdOutMin=[]  UintegralTsProdOutMax=[]  UngainTsProdOutMin=[]  UngainTsProdOutMax=[]  ClampingZeroOutDataTypeStr=Inherit: Inherit via back propagation  ClampingZeroOutMin=[]  ClampingZeroOutMax=[]  FilterDenConstantOutDataTypeStr=Inherit: Inherit via back propagation  FilterDenConstantOutMin=[]  FilterDenConstantOutMax=[]  PCopyOutDataTypeStr=Inherit: Inherit via back propagation  PCopyOutMin=[]  PCopyOutMax=[]  NCopyOutDataTypeStr=Inherit: Inherit via back propagation  NCopyOutMin=[]  NCopyOutMax=[]  IntegratorContinuousStateAttributes=''  IntegratorStateMustResolveToSignalObject=off  IntegratorRTWStateStorageClass=Auto  FilterContinuousStateAttributes=''  FilterStateMustResolveToSignalObject=off  FilterRTWStateStorageClass=Auto  ParallelPVariant=InternalParameters  IdealPVariant=Disabled  IVariant=InternalParameters  DVariant=Disabled  IntegratorVariant=Discrete  SatVariant=Disabled  AWVariant=Passthrough  PCopyVariant=Disabled  TRVariant=Disabled  FdbkBlocksVariant=Forward  IdealPFdbkVariant=Disabled  SatFdbkVariant=Disabled  DerivativeFilterVariant=Disabled  NVariant=Disabled  NCopyVariant=Disabled_SignalSpec  FilterICVariant=Disabled  IntegratorICVariant=InternalICs  ExternalResetVariant=Disabled  TRSumVariant=Passthrough  SumFdbkVariant=Disabled  SumVariant=Sum_PI  TsampFilterVariant=InternalTs  TsampNgainVariant=Passthrough  TsampIntegralVariant=Disabled_SignalSpec  ExternalSaturationOutDataTypeStr=Inherit: Same as second input  DerivativeSourceVariant=Disabled  PreIntVariant=InternalPreInt
  PID Controller1 : slpidlib/PID Controller  Controller=PI  Form=Parallel  TimeDomain=Discrete-time  UseExternalTs=off  SampleTime=-1  IntegratorMethod=Forward Euler  FilterMethod=Forward Euler  ControllerParametersSource=internal  P=P.ctrl.KpV  I=P.ctrl.KiV  UseKiTs=off  D=0  UseExternalDerivativeSource=off  N=100  UseFilter=on  TunerSelectOption=Transfer Function Based (PID Tuner App)  InitialConditionSource=internal  InitialConditionForIntegrator=0  InitialConditionForFilter=0  DifferentiatorICPrevScaledInput=0  ExternalReset=none  TrackingMode=off  Kt=1  LimitOutput=on  SatLimitsSource=internal  UpperSaturationLimit=P.ctrl.Ilim  LowerSaturationLimit=-P.ctrl.Ilim  LinearizeAsGain=on  AntiWindupMode=clamping  Kb=1  LimitIntegrator=off  UpperIntegratorSaturationLimit=inf  LowerIntegratorSaturationLimit=-inf  POutMin=[]  POutMax=[]  IOutMin=[]  IOutMax=[]  DOutMin=[]  DOutMax=[]  NOutMin=[]  NOutMax=[]  SumOutMin=[]  SumOutMax=[]  SaturationOutMin=[]  SaturationOutMax=[]  PParamMin=[]  PParamMax=[]  IParamMin=[]  IParamMax=[]  DParamMin=[]  DParamMax=[]  NParamMin=[]  NParamMax=[]  KbParamMin=[]  KbParamMax=[]  KtParamMin=[]  KtParamMax=[]  KbOutMin=[]  KbOutMax=[]  KtOutMin=[]  KtOutMax=[]  IntegratorOutMin=[]  IntegratorOutMax=[]  FilterOutMin=[]  FilterOutMax=[]  SumI1OutMin=[]  SumI1OutMax=[]  SumI2OutMin=[]  SumI2OutMax=[]  SumI3OutMin=[]  SumI3OutMax=[]  SumI4OutMin=[]  SumI4OutMax=[]  SumDOutMin=[]  SumDOutMax=[]  DifferentiatorOutMin=[]  DifferentiatorOutMax=[]  FilterDiffOutCoefMin=[]  FilterDiffOutCoefMax=[]  ReciprocalOutMin=[]  ReciprocalOutMax=[]  SumDenOutMin=[]  SumDenOutMax=[]  SumNumOutMin=[]  SumNumOutMax=[]  DivideOutMin=[]  DivideOutMax=[]  UdiffTsProdOutMin=[]  UdiffTsProdOutMax=[]  NTsProdOutMin=[]  NTsProdOutMax=[]  UintegralTsProdOutMin=[]  UintegralTsProdOutMax=[]  UngainTsProdOutMin=[]  UngainTsProdOutMax=[]  ClampingZeroOutDataTypeStr=Inherit: Inherit via back propagation  ClampingZeroOutMin=[]  ClampingZeroOutMax=[]  FilterDenConstantOutDataTypeStr=Inherit: Inherit via back propagation  FilterDenConstantOutMin=[]  FilterDenConstantOutMax=[]  PCopyOutDataTypeStr=Inherit: Inherit via back propagation  PCopyOutMin=[]  PCopyOutMax=[]  NCopyOutDataTypeStr=Inherit: Inherit via back propagation  NCopyOutMin=[]  NCopyOutMax=[]  IntegratorContinuousStateAttributes=''  IntegratorStateMustResolveToSignalObject=off  IntegratorRTWStateStorageClass=Auto  FilterContinuousStateAttributes=''  FilterStateMustResolveToSignalObject=off  FilterRTWStateStorageClass=Auto  ParallelPVariant=InternalParameters  IdealPVariant=Disabled  IVariant=InternalParameters  DVariant=Disabled  IntegratorVariant=Discrete  SatVariant=Enabled  AWVariant=DiscClampingParallel  PCopyVariant=Disabled  TRVariant=Disabled  FdbkBlocksVariant=Forward  IdealPFdbkVariant=Disabled  SatFdbkVariant=Disabled  DerivativeFilterVariant=Disabled  NVariant=Disabled  NCopyVariant=Disabled_SignalSpec  FilterICVariant=Disabled  IntegratorICVariant=InternalICs  ExternalResetVariant=Disabled  TRSumVariant=Passthrough  SumFdbkVariant=Disabled  SumVariant=Sum_PI  TsampFilterVariant=InternalTs  TsampNgainVariant=Passthrough  TsampIntegralVariant=Disabled_SignalSpec  ExternalSaturationOutDataTypeStr=Inherit: Same as second input  DerivativeSourceVariant=Disabled  PreIntVariant=InternalPreInt
  Saturation : Saturate  UpperLimit=1500  LowerLimit=50
  Saturation1 : Saturate  UpperLimit=1500  LowerLimit=50
  Scope5 : Scope  NumInputPorts=2
  Scope6 : Scope
  Selector : Selector  InputPortWidth=3  IndexOptions=Index vector (dialog)  Indices=2  OutputSizes=1
  Sum : Sum  Inputs=|-+
  Sum{1,4..6} (4 alike) : Sum  Inputs=|+-
  Sum2 : Sum  Inputs=|++
  Sum3 : Sum  Inputs=|++
  Sum7 : Sum  Inputs=|++
  Terminator : Terminator
  Terminator1 : Terminator
  abc to Alpha-Beta-Zero : spsabctoAlphaBetaZeroLib/abc to Alpha-Beta-Zero
  abc to dq0 : spsabctodq0Lib/abc to dq0  Alignment=90 degrees behind phase A axis
  dq0 to abc : spsdq0toabcLib/dq0 to abc  Alignment=90 degrees behind phase A axis
  rad_s to Hz : Gain  Gain=1/(2*pi)
  Vabc : Outport  VectorParamsAs1DForOutWhenUnconnected=off
  tag scope: ID=global, IQ=global, VD=global, VQ=global, alphabeta=global, freq=global, wt=global
  wires:
  Demux1/2 -> [VQ]
  Sum4/1 -> PID Controller1/1
  Constant3/1 -> Sum4/1
  Mux/1 -> dq0 to abc/1
  Sum2/1 -> Sum3/1
  [alphabeta] -> Alpha-Beta-Zero to dq1/1
  [VDC] -> Saturation/1
  [ID] -> Gain2/1
  Gain1/1 -> Divide/1
  Demux2/3 -> Terminator1/1
  PID Controller1/1 -> Gain4/1
  Divide1/1 -> Mux/2
  Gain4/1 -> Sum5/1
  Selector/1 -> Sum/1
  Saturation1/1 -> Divide1/2
  [wt] -> dq0 to abc/2
  PID Controller/1 -> Integrator/1, rad_s to Hz/1
  Demux1/3 -> Terminator/1
  Integrator/1 -> [wt], Alpha-Beta-Zero to dq1/2
  Constant2/1 -> Sum/2
  Sum/1 -> PID Controller/1
  abc to Alpha-Beta-Zero/1 -> [alphabeta], Alpha-Beta-Zero to dq0/1
  Divide/1 -> Mux/1
  dq0 to abc/1 -> Vabc/1, Scope6/1
  Gain/1 -> Sum6/2
  Demux1/1 -> [VD]
  Alpha-Beta-Zero to dq0/1 -> Demux1/1
  [VQ] -> Sum3/2
  Sum6/1 -> Sum7/1
  [VDC] -> Saturation1/1
  Alpha-Beta-Zero to dq1/1 -> Selector/1
  Sum7/1 -> Gain1/1
  [VD] -> Sum7/2
  [IQ] -> Sum1/2
  abc to dq0/1 -> Demux2/1
  [IQ] -> Gain/1
  Saturation/1 -> Divide/2
  Demux2/1 -> [ID]
  Sum3/1 -> Gain3/1
  [wt] -> Alpha-Beta-Zero to dq0/2
  [Iabc] -> abc to dq0/1
  [wt] -> abc to dq0/2
  Gain2/1 -> Sum2/2
  Gain3/1 -> Divide1/1
  Constant4/1 -> Mux/3
  Demux2/2 -> [IQ]
  [ID] -> Sum5/2
  [IQ] -> Scope5/1
  [Vabc] -> abc to Alpha-Beta-Zero/1
  [VDC] -> Sum4/2
  Sum5/1 -> Current controller d/1(error)
  Current controller d/1(u) -> Sum6/1
  Sum1/1 -> Current controller q/1(error)
  Current controller q/1(u) -> Scope5/2, Sum2/1
  Active frequency drift/1(Iq ref) -> Sum1/1
  rad_s to Hz/1 -> Frequency filter/1
  Frequency filter/1 -> Cycle mean/1
  Cycle mean/1 -> [freq]
